simulink model "LQG"  (R2024a)
settings: Solver=FixedStepAuto  StartTime=0.0  StopTime=Ts*2000  FixedStep=Ts  RelTol=1e-3
undefined symbols (not defined in the file): DiscIntNeverNeededParam, KLQRi, r, sys, Ts, x0
libraries: simulink x2
settings Model: Creator=wolf6845  LastModifiedBy=wolf6845
settings OptimizationCC: DefaultParameterBehavior=Inlined  UseDivisionForNetSlopeComputation=on  GainParamInheritBuiltInType=on  UseFloatMulNetSlope=on  InlineInvariantSignals=on  EfficientFloat2IntCast=on  LifeSpan=1  OptimizeDataStoreBuffers=off  BusAssignmentInplaceUpdate=off
settings DebuggingCC: SFUnexpectedBacktrackingDiag=warning  SFNoUnconditionalDefaultTransitionDiag=warning
settings HardwareCC: ProdLongLongMode=on
settings SFSimCC: MATLABDynamicMemAlloc=off
settings RTWCC: GenerateReport=on  BuildConfiguration=Debug  LaunchReport=on  GPUComputeCapability=3.5
settings CodeAppCC: ForceParamTrailComments=on  EnableCustomComments=on
settings GRTTargetCC: CombineSignalStateStructs=on  MatFileLogging=off  SupportVariableSizeSignals=on  MultiInstanceErrorCode=Warning

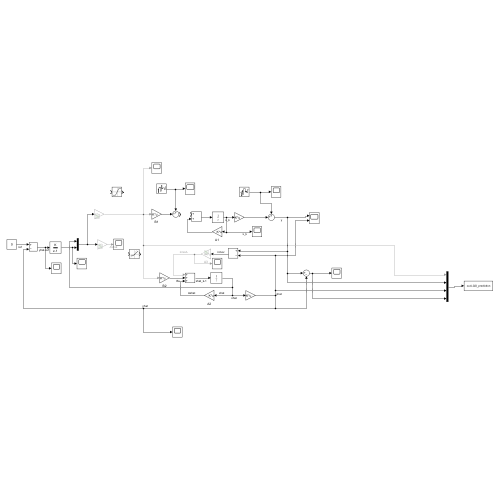
[thumbnail: Simulink's stored preview of the top-level diagram]
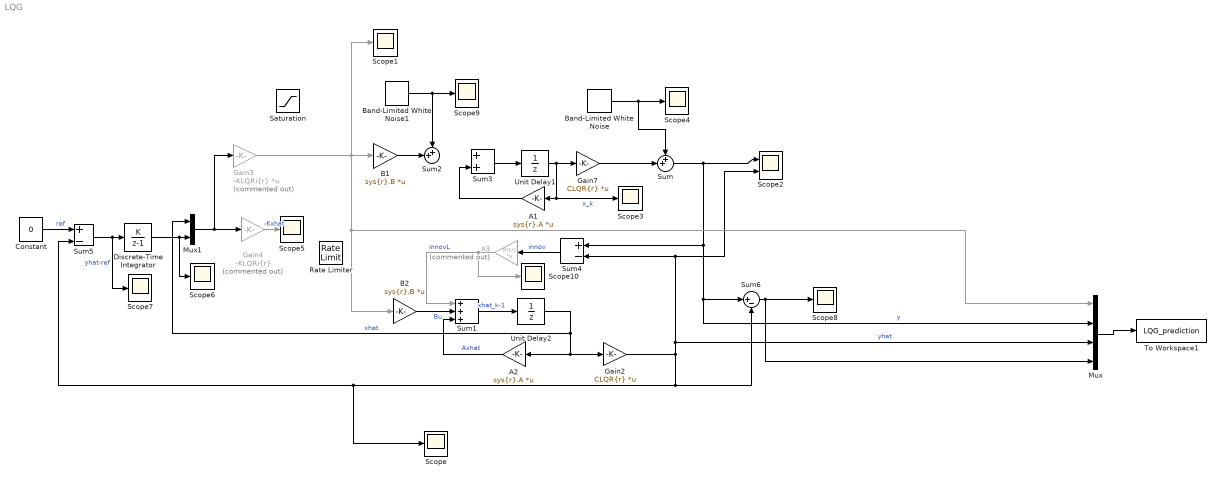
== system LQG ==
  A1 : Gain  Gain=sys{r}.A  Multiplication=Matrix(K*u)
  A2 : Gain  Gain=sys{r}.A  Multiplication=Matrix(K*u)
  A3 : Gain  Commented=on  Gain=Kf{r}  Multiplication=Matrix(K*u)
  B1 : Gain  Gain=sys{r}.B  Multiplication=Matrix(K*u)
  B2 : Gain  Gain=sys{r}.B  Multiplication=Matrix(K*u)
  Band-Limited White Noise : simulink/Sources/Band-Limited White Noise  Cov=0  Ts=Ts  seed=[23341]
  Band-Limited White Noise1 : simulink/Sources/Band-Limited White Noise  Cov=0  Ts=Ts*10  seed=[623087]
  Constant : Constant  Value=0
  Discrete-Time Integrator : DiscreteIntegrator  IntegratorMethod=Accumulation: Forward Euler  SampleTime=-1  ICPrevOutput=DiscIntNeverNeededParam  ICPrevScaledInput=DiscIntNeverNeededParam
  Gain2 : Gain  Gain=CLQR{r}  Multiplication=Matrix(K*u)
  Gain3 : Gain  Commented=on  Gain=-KLQRi{r}  Multiplication=Matrix(K*u)
  Gain4 : Gain  Commented=on  Gain=-KLQRi{r}
  Gain7 : Gain  Gain=CLQR{r}  Multiplication=Matrix(K*u)
  Mux : Mux
  Mux1 : Mux  Inputs=2
  Rate Limiter : RateLimiter  RisingSlewLimit=1400*80  FallingSlewLimit=-1400*80  SampleTimeMode=inherited
  Saturation : Saturate  UpperLimit=15  LowerLimit=-15
  Scope{,1,3..10} (10 alike) : Scope
  Scope2 : Scope  NumInputPorts=2
  Sum : Sum  Inputs=++|
  Sum1 : Sum  Inputs=+++
  Sum2 : Sum  Inputs=++|
  Sum3 : Sum
  Sum4 : Sum  Inputs=+-
  Sum5 : Sum  Inputs=+-
  Sum6 : Sum  Inputs=|+-
  To Workspace1 : ToWorkspace  VariableName=LQG_prediction  SampleTime=-1
      settings: Save2DSignal=2-D array (concatenate along first dimension)
  Unit Delay1 : UnitDelay  InitialCondition=x0(1:size(sys{r}.A,1))  SampleTime=Ts  HasFrameUpgradeWarning=on
  Unit Delay2 : UnitDelay  SampleTime=Ts  HasFrameUpgradeWarning=on
  wires:
  A1/1 -> Sum3/2
  Constant/1 -> Sum5/1  "ref"
  A2/1 -> Sum1/3  "Axhat"
  Sum4/1 -> A3/1  "innov"
  Sum1/1 -> Unit Delay2/1  "xhat_k-1"
  Sum3/1 -> Unit Delay1/1
  A3/1 -> Scope10/1, Sum1/1  "innovL"
  B2/1 -> Sum1/2  "Bu"
  Unit Delay1/1 -> Scope3/1, A1/1, Gain7/1  "x_k"
  Band-Limited White Noise/1 -> Sum/1, Scope4/1
  Sum5/1 -> Scope7/1, Discrete-Time Integrator/1  "yhat-ref"
  Sum/1 -> Mux/2, Sum6/1, Sum4/1, Scope2/1  "y"
  Gain2/1 -> Scope2/2, Sum4/2, Mux/3, Scope/1, Sum5/2, Sum6/2  "yhat"
  Sum6/1 -> Mux/4, Scope8/1
  Unit Delay2/1 -> Gain2/1, A2/1, Mux1/1  "xhat"
  Mux1/1 -> Gain3/1, Gain4/1
  Gain4/1 -> Scope5/1  "-Kxhat"
  Mux/1 -> To Workspace1/1
  Discrete-Time Integrator/1 -> Scope6/1, Mux1/2
  Band-Limited White Noise1/1 -> Sum2/1, Scope9/1
  Gain3/1 -> B1/1, Mux/1, B2/1, Scope1/1
  Gain7/1 -> Sum/2
  B1/1 -> Sum2/2
